simulink model "ann_transmission_line"  (R2024a)
settings: Solver=FixedStepDiscrete  StartTime=0.0  StopTime=0.26  FixedStep=5.0000000000000002e-05  RelTol=1e-3
libraries: spsThreePhasePISectionLineLib x2, spsThreePhaseFaultLib x1, spsThreePhaseParallelRLCLoadLib x1, spsThreePhaseVIMeasurementLib x1, spsThreePhaseSourceLib x1, spsThreePhaseTransformerTwoWindingsLib x1, spspowerguiLib x1
settings Model: Creator=crack  LastModifiedBy=crack

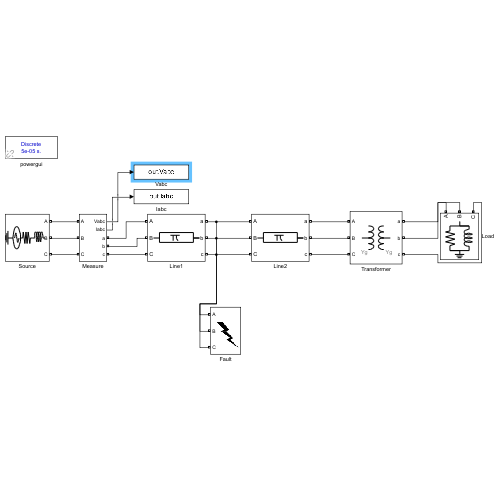
[thumbnail: Simulink's stored preview of the top-level diagram]
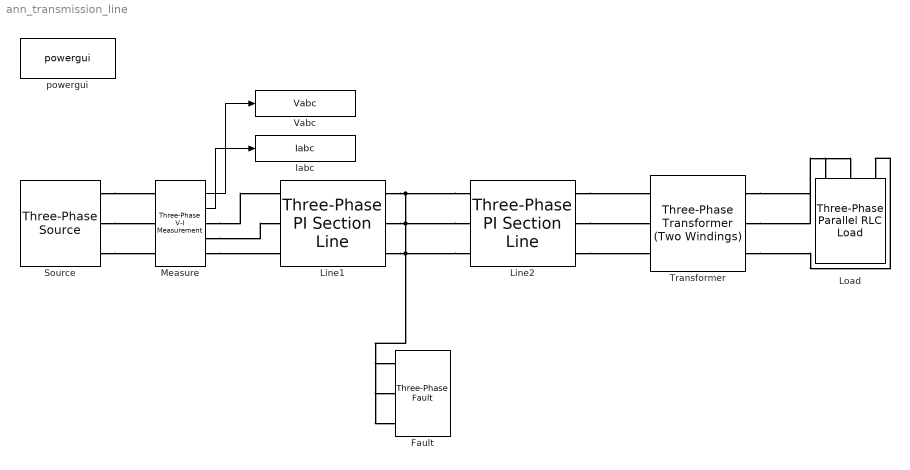
== system ann_transmission_line ==
  Fault : spsThreePhaseFaultLib/Three-Phase Fault  InitialStates=0  FaultA=on  FaultB=off  FaultC=off  GroundFault=on  SwitchTimes=[0.1 0.3]  External=off  SwitchStatus=NaN  FaultResistance=0.1  GroundResistance=0.1  SnubberResistance=1e6  SnubberCapacitance=inf  Measurements=None
  Iabc : ToWorkspace  VariableName=Iabc  SaveFormat=Timeseries  SampleTime=-1
  Line1 : spsThreePhasePISectionLineLib/Three-Phase PI Section Line  LConnTagsString=a|b|c  RConnTagsString=A|B|C  Length=5  Frequency=50  Resistances=[0.01273 0.38640000000000002]  Inductances=[0.00093369999999999998 0.0041263999999999997]  Capacitances=[1.274e-08 7.7509999999999994e-09]
  Line2 : spsThreePhasePISectionLineLib/Three-Phase PI Section Line  LConnTagsString=a|b|c  RConnTagsString=A|B|C  Length=5  Frequency=50  Resistances=[0.01273 0.38640000000000002]  Inductances=[0.00093369999999999998 0.0041263999999999997]  Capacitances=[1.274e-08 7.7509999999999994e-09]
  Load : spsThreePhaseParallelRLCLoadLib/Three-Phase Parallel RLC Load  LConnTagsString=A|B|C  Configuration=Y (grounded)  NominalVoltage=400  Vabc=[1e3 1e3 1e3]  Vabcp=[1e3 1e3 1e3]  NominalFrequency=50  UnbalancedPower=off  ActivePower=800000  InductivePower=300000  CapacitivePower=0  Pabc=[10e3 9e3 11e3]  QLabc=[100 90 110]  QCabc=[100 90 110]  Pabcp=[10e3 9e3 11e3]  QLabcp=[100 90 110]  QCabcp=[100 90 110]  Measurements=None  LoadType=constant Z
  Measure : spsThreePhaseVIMeasurementLib/Three-Phase V-I Measurement  VoltageMeasurement=phase-to-ground  SetLabelV=off  LabelV=Vabc  Vpu=off  VpuLL=off  CurrentMeasurement=yes  SetLabelI=off  LabelI=Iabc  Ipu=off  Pbase=100e6  Vbase=500e3  OutputType=Complex  PhasorSimulation=off  PSBequivalent=0
  Source : spsThreePhaseSourceLib/Three-Phase Source  InternalConnection=Yg  VoltagePhases=off  Voltage=11000  PhaseAngle=0  Voltage_phases=[25e3 25e3 25e3]/sqrt(3)  PhaseAngles_phases=[0 -120 +120]  Frequency=50  NonIdealSource=on  SpecifyImpedance=off  Resistance=4.0331316817904064  Inductance=0.00012837856865949445  ShortCircuitLevel=100e6  BaseVoltage=25e3  XRratio=7  BusType=swing  Pref=10e3  Qref=0  Prefabc=[10e3, 10e3, 10e3]  Qrefabc=[0, 0, 0]  Qmin=-inf  Qmax=inf
  Transformer : spsThreePhaseTransformerTwoWindingsLib/Three-Phase Transformer (Two Windings)  Winding1Connection=Yg  Winding2Connection=Yg  CoreType=Three single-phase transformers  SetSaturation=off  Hysteresis=off  DataFile='hysteresis'  SetInitialFlux=off  Measurements=None  UNITS=pu  NominalPower=[1e6 50]  Winding1=[11000 0.005 0.025]  Winding2=[400 0.005 0.025]  Rm=500  Lm=500  L0=0.5  Saturation=[ 0,0 ; 0.0024,1.2 ; 1.0,1.52 ]  InitialFluxes=[ 0.8 , -0.8 , 0.7 ]  BreakLoop=off  DiscreteSolver=Trapezoidal iterative  DataType=off  TransfoNumber=1
  Vabc : ToWorkspace  VariableName=Vabc  SaveFormat=Timeseries  SampleTime=-1
  powergui : spspowerguiLib/powergui  Priority=1  SimulationMode=Discrete  SampleTime=5.0000000000000002e-05  frequency=60  Iterations=50  frequencyindice=50  Pbase=100e6  ErrMax=1e-4  UnitsV=kV  UnitsW=MW  buscounter=0  FunctionMessages=off  echomessages=off  EnableUseOfTLC=off  CurrentSourceSwitches=off  DisableSnubberDevices=off  DisableRonSwitches=off  DisableVfSwitches=off  DisplayEquations=off  AutomaticDiscreteSolvers=off  SolverType=Tustin/Backward Euler (TBE)  Interpol=off  ExternalGateDelay=off  methode=off  Ts=100  x0status=blocks  SPID=on  SwTol=0  HookPort=off  NonlinearTolerance=1e-4  nMaxIteration=100  ContinueOnMaxIteration=off  RestoreLinks=warning  ResistiveCurrentMeasurement=off  Frange=[0:2:500]  Ylog=off  Xlog=on  ShowGrid=off  save=off  variable=ZData  structure=0  ZoomFFT=off  StartTime=0.0  cycles=1  DisplayStyle=1  fundamental=60  FreqAxis=off  MaxFrequency=1000  frequencyindicesteady=1  RmsSteady=1  display=off
  wires:
  Measure/1 -> Vabc/1
  Measure/2 -> Iabc/1
  connections:
  Source/RConn1 -- Measure/LConn1
  Source/RConn2 -- Measure/LConn2
  Source/RConn3 -- Measure/LConn3
  Measure/RConn1 -- Line1/LConn1
  Measure/RConn2 -- Line1/LConn2
  Measure/RConn3 -- Line1/LConn3
  Line2/LConn1 -- Line1/RConn1 -- Fault/LConn1
  Line2/LConn2 -- Line1/RConn2 -- Fault/LConn2
  Line2/LConn3 -- Line1/RConn3 -- Fault/LConn3
  Line2/RConn1 -- Transformer/LConn1
  Line2/RConn2 -- Transformer/LConn2
  Line2/RConn3 -- Transformer/LConn3
  Transformer/RConn1 -- Load/LConn1
  Transformer/RConn2 -- Load/LConn2
  Transformer/RConn3 -- Load/LConn3
